simulink model "afe_rst_inv_psm_distributed_control_two_delays"  (R2026a)
settings: Solver=ode1be  StopTime=simlength  FixedStep=tc  MaxStep=Tc
values from neighbouring files (symbols this model uses):
  Amplitude_U = 1.16    [grid_fault_generator.m]
  Amplitude_V = Amplitude_U    (= 1.16)    [grid_fault_generator.m]
  Amplitude_W = Amplitude_U    (= 1.16)    [grid_fault_generator.m]
  end_time_LVRT = start_time_LVRT + error_length    [grid_fault_generator.m]
  Igrid_phase_normalization_factor = 270*sqrt(2)    [grid_emulator.m]
  omega_grid_emulator_nom = w_grid    (= 314.159265359)    [grid_emulator.m]
  omega_grid_nom = w_grid    (= 314.159265359)    [grid_emulator.m]
  t_ramp = 20e-3    (= 0.02)    [grid_fault_generator.m]
  ugrid_factor = 1    [grid_emulator.m]
  V_phase_normalization_factor = Vgrid_phase_normalization_factor    [grid_emulator.m]
  Vdc_bez = 1070    [grid_emulator.m]
  Vemu_ref_norm = Vemu_ref * sqrt(2) / V_phase_normalization_factor    [grid_emulator.m]
  vn_eta_pu = 0    [grid_emulator.m]
  vn_xi_pu = 0    [grid_emulator.m]
  vp_xi_pu = 1    [grid_emulator.m]
undefined symbols (not defined in the file or in its folder): Adrso, Aresd, Bresd, CFi, CFu, Cresd, Crso, CTRPIFF_CLIP_RELEASE, dead_time_INV, emf_fb_p, emf_fb_p_ccaller_1, emf_fb_p_ccaller_2, emf_p, emf_p_ccaller_1, emf_p_ccaller_2, fPWM_INV, g0_161Hz, g0_500Hz, g1_161Hz, g1_500Hz, i_grid_neg_eta_lim, i_grid_neg_eta_red_lim, i_grid_neg_xi_lim, i_grid_neg_xi_red_lim, i_grid_pos_eta_lim, i_grid_pos_eta_red_lim, ibez, id_lim, ieta_neg_ref_lim, ieta_pos_ref_lim, iq_lim, ixi_pos_ref_lim, Jm_norm, k_frt_ref, kg, ki_afe, ki_i, ki_id, ki_iq, ki_rc_neg_grid, ki_rc_pos_grid, ki_vs, ki_w, kp_afe, kp_i, kp_id, kp_iq, kp_rc_neg_grid, kp_rc_pos_grid, kp_vs, kp_w, kw, l1, l2, Lalpha_norm, Ld_norm, Ldrso, Lq_norm, Ls_norm, luenberger_l1 ... (+30)
libraries: fl_lib x146, nesl_utility x62, simulink x8, cstblocks_lti x7, sl_discontinuities x3, single_phase_transformer_lib x3, flexshaft_lib x1, permanent_magnet_synchronous_machine x1
(part 9 of 14)

== system afe_rst_inv_psm_distributed_control_two_delays/INV-Modular/inv_leg_w/driver_board_w/voltage-current-acquisition/usu_fieldbus ==
  us : Inport
  Unit Delay : UnitDelay  SampleTime=ts_inv
  Unit Delay1 : UnitDelay  SampleTime=ts_inv
  Zero-Order Hold : ZeroOrderHold  SampleTime=ts_inv
  us_fb : Outport
  wires:
  Zero-Order Hold/1 -> Unit Delay/1
  us/1 -> Zero-Order Hold/1
  Unit Delay/1 -> Unit Delay1/1
  Unit Delay1/1 -> us_fb/1

== system afe_rst_inv_psm_distributed_control_two_delays/INV-Modular/inv_leg_w/driver_board_w/voltage-current-acquisition/usv_ctrl_fieldbus ==
  u_ctrl : Inport
  Unit Delay : UnitDelay  SampleTime=ts_inv
  Unit Delay1 : UnitDelay  SampleTime=ts_inv
  Zero-Order Hold : ZeroOrderHold  SampleTime=ts_inv
  u_ctrl_fb : Outport
  wires:
  Zero-Order Hold/1 -> Unit Delay/1
  u_ctrl/1 -> Zero-Order Hold/1
  Unit Delay/1 -> Unit Delay1/1
  Unit Delay1/1 -> u_ctrl_fb/1

== system afe_rst_inv_psm_distributed_control_two_delays/INV-Modular/inv_leg_w/driver_board_w/voltage-current-acquisition/usv_fieldbus ==
  us : Inport
  Unit Delay : UnitDelay  SampleTime=ts_inv
  Unit Delay1 : UnitDelay  SampleTime=ts_inv
  Zero-Order Hold : ZeroOrderHold  SampleTime=ts_inv
  us_fb : Outport
  wires:
  Zero-Order Hold/1 -> Unit Delay/1
  us/1 -> Zero-Order Hold/1
  Unit Delay/1 -> Unit Delay1/1
  Unit Delay1/1 -> us_fb/1

== system afe_rst_inv_psm_distributed_control_two_delays/INV-Modular/inv_leg_w/driver_board_w/voltage-current-acquisition/usw_measure_and_normalization ==
  us : Inport
  Gain : Gain  Gain=1/ubez
  Quantizer : Quantizer  QuantizationInterval=CurrentQuantization
  Unit Delay : UnitDelay  SampleTime=ts_afe
  Zero-Order Hold : ZeroOrderHold  SampleTime=ts_afe
  us_pu : Outport
  wires:
  Quantizer/1 -> Zero-Order Hold/1
  Gain/1 -> us_pu/1
  Zero-Order Hold/1 -> Unit Delay/1
  Unit Delay/1 -> Gain/1
  us/1 -> Quantizer/1

== system afe_rst_inv_psm_distributed_control_two_delays/INV-Modular/inv_leg_w/modulator/sv_pwm/modulator ==
  w : Inport
  Bus Creator : BusCreator  Inputs=2
  PWM generator : Subsystem  mask{f=fPWM_INV, ph=0, m_up=0.98, m_low=0.02, dead_time=dead_time_INV, vg_firing=15, polarity=1}
      mask prompts: f "Frequency"; ph "Phase"; m_up "Max Input Modulation Value"; m_low "Min Input Modulation Value"; dead_time "Dead Time"; vg_firing "Gate Voltage"
  firing_gates : Outport
  wires:
  PWM generator/2(m2) -> Bus Creator/2  "pwm_w_bottom"
  PWM generator/1(m1) -> Bus Creator/1  "pwm_w_top"
  Bus Creator/1 -> firing_gates/1
  w/1 -> PWM generator/1(m_index)

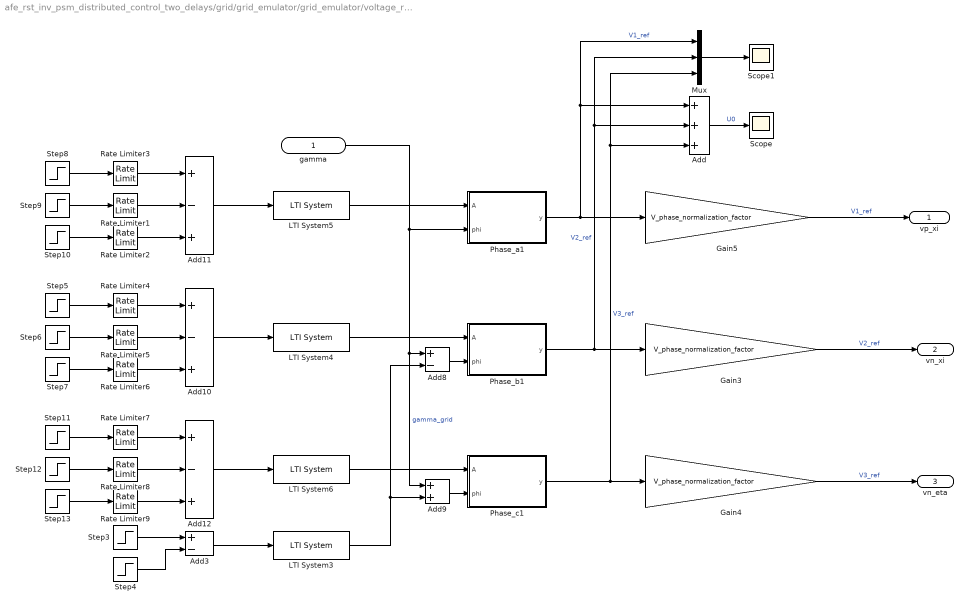
== system afe_rst_inv_psm_distributed_control_two_delays/grid/grid_emulator/grid_emulator/voltage_reference/Grid: Voltage-Source in abc ==
  gamma : Inport
  Add : Sum  Inputs=+++
  Add10 : Sum  Inputs=+-+
  Add11 : Sum  Inputs=+-+
  Add12 : Sum  Inputs=+-+
  Add3 : Sum  Inputs=+-
  Add8 : Sum  Inputs=+-
  Add9 : Sum
  Gain3 : Gain  Gain=V_phase_normalization_factor
  Gain4 : Gain  Gain=V_phase_normalization_factor
  Gain5 : Gain  Gain=V_phase_normalization_factor
  LTI System{3..6} (4 alike) : cstblocks_lti/LTI System  sys=LVRT_flt_ss_c  IC=[0]  PadeOrder=0
  Mux : Mux  Inputs=3
  Phase_a1 : MATLAB Function  TreatAsAtomicUnit=on
  Phase_b1 : MATLAB Function  TreatAsAtomicUnit=on
  Phase_c1 : MATLAB Function  TreatAsAtomicUnit=on
  Rate Limiter{1..9} (9 alike) : RateLimiter  RisingSlewLimit=Vemu_ref_norm/t_ramp  FallingSlewLimit=-Vemu_ref_norm/t_ramp  SampleTimeMode=inherited
  Scope : Scope
      settings: SampleTime=tc  ActiveDisplayYMinimum=-1.1E-15  ActiveDisplayYMaximum=9E-16
  Scope1 : Scope
      settings: SampleTime=tc  ActiveDisplayYMinimum=-1.24491  ActiveDisplayYMaximum=1.24491
  Step10 : Step  Time=end_time_LVRT  FinalValue=Vemu_ref_norm*(1-Amplitude_U)  SampleTime=0
  Step11 : Step  Time=0  FinalValue=Vemu_ref_norm  SampleTime=0
  Step12 : Step  Time=start_time_LVRT  FinalValue=Vemu_ref_norm*(1-Amplitude_W)  SampleTime=0
  Step13 : Step  Time=end_time_LVRT  FinalValue=Vemu_ref_norm*(1-Amplitude_W)  SampleTime=0
  Step3 : Step  Time=start_time_LVRT  FinalValue=Phase_shift  SampleTime=0
  Step4 : Step  Time=end_time_LVRT  FinalValue=Phase_shift  SampleTime=0
  Step5 : Step  Time=0  FinalValue=Vemu_ref_norm  SampleTime=0
  Step6 : Step  Time=start_time_LVRT  FinalValue=Vemu_ref_norm*(1-Amplitude_V)  SampleTime=0
  Step7 : Step  Time=end_time_LVRT  FinalValue=Vemu_ref_norm*(1-Amplitude_V)  SampleTime=0
  Step8 : Step  Time=0  FinalValue=Vemu_ref_norm  SampleTime=0
  Step9 : Step  Time=start_time_LVRT  FinalValue=Vemu_ref_norm*(1-Amplitude_U)  SampleTime=0
  vp_xi : Outport  VectorParamsAs1DForOutWhenUnconnected=off
  vn_xi : Outport  Port=2  VectorParamsAs1DForOutWhenUnconnected=off
  vn_eta : Outport  Port=3  VectorParamsAs1DForOutWhenUnconnected=off
  wires:
  Phase_c1/1(y) -> Mux/3, Add/3, Gain4/1  "V3_ref"
  LTI System6/1 -> Phase_c1/1(A)
  gamma/1 -> Add9/1, Add8/1, Phase_a1/2(phi)  "gamma_grid"
  Add9/1 -> Phase_c1/2(phi)
  Add8/1 -> Phase_b1/2(phi)
  Phase_b1/1(y) -> Mux/2, Add/2, Gain3/1  "V2_ref"
  Phase_a1/1(y) -> Mux/1, Add/1, Gain5/1  "V1_ref"
  LTI System4/1 -> Phase_b1/1(A)
  Step5/1 -> Rate Limiter4/1
  Step6/1 -> Rate Limiter5/1
  Step7/1 -> Rate Limiter6/1
  Add10/1 -> LTI System4/1
  Step8/1 -> Rate Limiter3/1
  Add11/1 -> LTI System5/1
  Step9/1 -> Rate Limiter1/1
  Step10/1 -> Rate Limiter2/1
  LTI System5/1 -> Phase_a1/1(A)
  Add12/1 -> LTI System6/1
  Rate Limiter3/1 -> Add11/1
  Rate Limiter1/1 -> Add11/2
  Rate Limiter2/1 -> Add11/3
  Rate Limiter4/1 -> Add10/1
  Rate Limiter5/1 -> Add10/2
  Rate Limiter6/1 -> Add10/3
  Step12/1 -> Rate Limiter8/1
  Rate Limiter8/1 -> Add12/2
  Step13/1 -> Rate Limiter9/1
  Rate Limiter9/1 -> Add12/3
  Step11/1 -> Rate Limiter7/1
  Rate Limiter7/1 -> Add12/1
  Gain5/1 -> vp_xi/1  "V1_ref"
  Gain3/1 -> vn_xi/1  "V2_ref"
  Gain4/1 -> vn_eta/1  "V3_ref"
  Add3/1 -> LTI System3/1
  Step3/1 -> Add3/1
  Step4/1 -> Add3/2
  LTI System3/1 -> Add9/2, Add8/2
  Add/1 -> Scope/1  "U0"
  Mux/1 -> Scope1/1

== system afe_rst_inv_psm_distributed_control_two_delays/mainboard_afe/dq_pll/pll_stageA/sequences/alphabeta2xieta ==
  alpha : Inport
  beta : Inport  Port=2
  gamma : Inport  Port=3
  alphabeta2xieta_neg : MATLAB Function  TreatAsAtomicUnit=on  SystemSampleTime=ts_afe
  alphabeta2xieta_pos : MATLAB Function  TreatAsAtomicUnit=on  SystemSampleTime=ts_afe
  xi : Outport
  eta : Outport  Port=2
  Out3 : Outport  Port=3
  Out4 : Outport  Port=4
  wires:
  alpha/1 -> alphabeta2xieta_neg/1(alpha), alphabeta2xieta_pos/1(alpha)  "u_grid_alpha"
  beta/1 -> alphabeta2xieta_neg/2(beta), alphabeta2xieta_pos/2(beta)  "u_grid_beta"
  gamma/1 -> alphabeta2xieta_neg/3(gamma), alphabeta2xieta_pos/3(gamma)  "gamma_grid"
  alphabeta2xieta_pos/1(xi) -> xi/1  "u_grid_pos_xi"
  alphabeta2xieta_pos/2(eta) -> eta/1  "u_grid_pos_eta"
  alphabeta2xieta_neg/1(xi) -> Out3/1  "u_grid_neg_xi"
  alphabeta2xieta_neg/2(eta) -> Out4/1  "u_grid_neg_eta"

== system afe_rst_inv_psm_distributed_control_two_delays/AFE-Modular/afe_leg_a/driver_board_a/current_ctrl/phase_current_control/phase-current-control-dba ==
  In1 : Inport
  is_abc : Inport  Port=2
  Add : Sum
  Add1 : Sum
  Cresd./Tcontrol new1 : Gain  Gain=Cresd  Multiplication=Matrix(K*u)
  Gain : Gain  Gain=kp_afe
  Gain1 : Gain  Gain=ki_afe
  Gain2 : Gain  Gain=Bresd  Multiplication=Matrix(K*u)
  Gain3 : Gain  Gain=Aresd  Multiplication=Matrix(K*u)
  Sum : Sum  Inputs=|+-
  Sum2 : Sum  Inputs=|++  SaturateOnIntegerOverflow=on
  Unit Delay : UnitDelay  InitialCondition=[0 0]  SampleTime=ts_afe
  Out1 : Outport
  wires:
  Cresd./Tcontrol new1/1 -> Add/2  "y(k)"
  Gain3/1 -> Sum2/2
  Sum2/1 -> Unit Delay/1  "x(k+1)"
  Unit Delay/1 -> Cresd./Tcontrol new1/1, Gain3/1  "x(k)"
  Gain2/1 -> Sum2/1
  Gain1/1 -> Gain2/1  "u(k)"
  Gain/1 -> Add/1
  Sum/1 -> Gain/1, Gain1/1
  is_abc/1 -> Sum/2  "isa"
  In1/1 -> Sum/1  "isa_ref"
  Add/1 -> Add1/1  "u_ctrl_a"
  [uga_pu_dba_flt] -> Add1/2
  Add1/1 -> Out1/1  "u_ctrl_a"

== system afe_rst_inv_psm_distributed_control_two_delays/AFE-Modular/afe_leg_a/driver_board_a/dq_pll/pll_stageA/sequences ==
  u_grid_alpha : Inport
  u_grid_beta : Inport  Port=2
  gamma_grid : Inport  Port=3
  alphabeta2xieta : Subsystem
  u_grid_pos_xi : Outport
  u_grid_pos_eta : Outport  Port=2
  wires:
  alphabeta2xieta/1(xi) -> u_grid_pos_xi/1  "u_grid_pos_xi"
  alphabeta2xieta/2(eta) -> u_grid_pos_eta/1  "u_grid_pos_eta"
  u_grid_alpha/1 -> alphabeta2xieta/1(alpha)  "u_grid_alpha"
  u_grid_beta/1 -> alphabeta2xieta/2(beta)  "u_grid_beta"
  gamma_grid/1 -> alphabeta2xieta/3(gamma)  "gamma_grid"

== system afe_rst_inv_psm_distributed_control_two_delays/AFE-Modular/afe_leg_a/driver_board_a/dq_pll/pll_stageA/transformation ==
  ug_a : Inport
  ug_b : Inport  Port=2
  ug_c : Inport  Port=3
  abc2alphabeta : MATLAB Function  TreatAsAtomicUnit=on  SystemSampleTime=ts_afe
  u_500Hz_flt : Subsystem
  ug_alpha : Outport  VectorParamsAs1DForOutWhenUnconnected=off
  ug_beta : Outport  Port=2  VectorParamsAs1DForOutWhenUnconnected=off
  tag scope: uga_pu_dba_flt=global
  wires:
  abc2alphabeta/2(beta) -> ug_beta/1  "u_grid_beta"
  abc2alphabeta/1(alpha) -> ug_alpha/1  "u_grid_alpha"
  ug_c/1 -> abc2alphabeta/3(c)
  ug_b/1 -> abc2alphabeta/2(b)
  u_500Hz_flt/1(output) -> [uga_pu_dba_flt]
  ug_a/1 -> u_500Hz_flt/1(input), abc2alphabeta/1(a)

== system afe_rst_inv_psm_distributed_control_two_delays/AFE-Modular/afe_leg_a/modulator/sv_pwm/modulator/PWM generator 1 ==
  m_index : Inport
  Constant : Constant  Value=dead_time*f
  Constant1 : Constant
  Data Type Conversion1 : DataTypeConversion
  Data Type Conversion2 : DataTypeConversion
  Gain : Gain  Gain=1/(pi/2)
  Gain1 : Gain  Gain=1/2
  Gain2 : Gain  Gain=vg_firing
  Gain3 : Gain  Gain=vg_firing
  Gain4 : Gain  Gain=polarity
  Gain5 : Gain  Gain=polarity
  Hit Crossing : HitCross  Commented=on  ShowOutputPort=off
  Hit Crossing1 : HitCross  Commented=on  ShowOutputPort=off
  Relational Operator1 : RelationalOperator  Operator=<=  InputSameDT=off
  Relational Operator2 : RelationalOperator  Operator=<=  InputSameDT=off
  Saturation1 : Saturate  UpperLimit=m_up  LowerLimit=m_low
  Sine Wave : Sin  Frequency=f*2*pi  Phase=-pi/2+ph  SampleTime=0
  Sum : Sum  Inputs=|++  SaturateOnIntegerOverflow=on
  Sum1 : Sum  Inputs=-+|  SaturateOnIntegerOverflow=on
  Sum2 : Sum  Inputs=|++
  Trigonometric Function1 : Trigonometry  Operator=asin
  m1 : Outport
  m2 : Outport  Port=2
  wires:
  Relational Operator1/1 -> Data Type Conversion1/1
  m_index/1 -> Saturation1/1
  Relational Operator2/1 -> Data Type Conversion2/1
  Data Type Conversion2/1 -> Gain3/1, Hit Crossing1/1
  Constant/1 -> Sum/2, Sum1/1
  Saturation1/1 -> Sum/1, Sum1/2
  Sum/1 -> Relational Operator1/1
  Sum1/1 -> Relational Operator2/2
  Sine Wave/1 -> Trigonometric Function1/1
  Constant1/1 -> Sum2/2
  Trigonometric Function1/1 -> Gain/1
  Gain/1 -> Sum2/1
  Sum2/1 -> Gain1/1
  Gain1/1 -> Relational Operator2/1, Relational Operator1/2
  Data Type Conversion1/1 -> Hit Crossing/1, Gain2/1
  Gain2/1 -> Gain4/1
  Gain3/1 -> Gain5/1
  Gain4/1 -> m1/1
  Gain5/1 -> m2/1

== system afe_rst_inv_psm_distributed_control_two_delays/AFE-Modular/afe_leg_a/modulator/sv_pwm/modulator/PWM generator 2 ==
  m_index : Inport
  Constant : Constant  Value=dead_time*f
  Constant1 : Constant
  Data Type Conversion1 : DataTypeConversion
  Data Type Conversion2 : DataTypeConversion
  Gain : Gain  Gain=1/(pi/2)
  Gain1 : Gain  Gain=1/2
  Gain2 : Gain  Gain=vg_firing
  Gain3 : Gain  Gain=vg_firing
  Gain4 : Gain  Gain=polarity
  Gain5 : Gain  Gain=polarity
  Hit Crossing : HitCross  Commented=on  ShowOutputPort=off
  Hit Crossing1 : HitCross  Commented=on  ShowOutputPort=off
  Relational Operator1 : RelationalOperator  Operator=<=  InputSameDT=off
  Relational Operator2 : RelationalOperator  Operator=<=  InputSameDT=off
  Saturation1 : Saturate  UpperLimit=m_up  LowerLimit=m_low
  Sine Wave : Sin  Frequency=f*2*pi  Phase=-pi/2+ph  SampleTime=0
  Sum : Sum  Inputs=|++  SaturateOnIntegerOverflow=on
  Sum1 : Sum  Inputs=-+|  SaturateOnIntegerOverflow=on
  Sum2 : Sum  Inputs=|++
  Trigonometric Function1 : Trigonometry  Operator=asin
  m1 : Outport
  m2 : Outport  Port=2
  wires:
  Gain5/1 -> m2/1
  Gain4/1 -> m1/1
  Gain3/1 -> Gain5/1
  Gain2/1 -> Gain4/1
  Data Type Conversion1/1 -> Gain2/1, Hit Crossing/1
  Gain1/1 -> Relational Operator1/2, Relational Operator2/1
  Sum2/1 -> Gain1/1
  Gain/1 -> Sum2/1
  Trigonometric Function1/1 -> Gain/1
  Constant1/1 -> Sum2/2
  Sine Wave/1 -> Trigonometric Function1/1
  Sum1/1 -> Relational Operator2/2
  Sum/1 -> Relational Operator1/1
  Saturation1/1 -> Sum1/2, Sum/1
  Constant/1 -> Sum1/1, Sum/2
  Data Type Conversion2/1 -> Hit Crossing1/1, Gain3/1
  Relational Operator2/1 -> Data Type Conversion2/1
  m_index/1 -> Saturation1/1
  Relational Operator1/1 -> Data Type Conversion1/1

== system afe_rst_inv_psm_distributed_control_two_delays/AFE-Modular/afe_leg_a/modulator/sv_pwm/modulator/PWM generator 3 ==
  m_index : Inport
  Constant : Constant  Value=dead_time*f
  Constant1 : Constant
  Data Type Conversion1 : DataTypeConversion
  Data Type Conversion2 : DataTypeConversion
  Gain : Gain  Gain=1/(pi/2)
  Gain1 : Gain  Gain=1/2
  Gain2 : Gain  Gain=vg_firing
  Gain3 : Gain  Gain=vg_firing
  Gain4 : Gain  Gain=polarity
  Gain5 : Gain  Gain=polarity
  Hit Crossing : HitCross  Commented=on  ShowOutputPort=off
  Hit Crossing1 : HitCross  Commented=on  ShowOutputPort=off
  Relational Operator1 : RelationalOperator  Operator=<=  InputSameDT=off
  Relational Operator2 : RelationalOperator  Operator=<=  InputSameDT=off
  Saturation1 : Saturate  UpperLimit=m_up  LowerLimit=m_low
  Sine Wave : Sin  Frequency=f*2*pi  Phase=-pi/2+ph  SampleTime=0
  Sum : Sum  Inputs=|++  SaturateOnIntegerOverflow=on
  Sum1 : Sum  Inputs=-+|  SaturateOnIntegerOverflow=on
  Sum2 : Sum  Inputs=|++
  Trigonometric Function1 : Trigonometry  Operator=asin
  m1 : Outport
  m2 : Outport  Port=2
  wires:
  Relational Operator1/1 -> Data Type Conversion1/1
  m_index/1 -> Saturation1/1
  Relational Operator2/1 -> Data Type Conversion2/1
  Data Type Conversion2/1 -> Gain3/1, Hit Crossing1/1
  Constant/1 -> Sum/2, Sum1/1
  Saturation1/1 -> Sum/1, Sum1/2
  Sum/1 -> Relational Operator1/1
  Sum1/1 -> Relational Operator2/2
  Sine Wave/1 -> Trigonometric Function1/1
  Constant1/1 -> Sum2/2
  Trigonometric Function1/1 -> Gain/1
  Gain/1 -> Sum2/1
  Sum2/1 -> Gain1/1
  Gain1/1 -> Relational Operator2/1, Relational Operator1/2
  Data Type Conversion1/1 -> Hit Crossing/1, Gain2/1
  Gain2/1 -> Gain4/1
  Gain3/1 -> Gain5/1
  Gain4/1 -> m1/1
  Gain5/1 -> m2/1

== system afe_rst_inv_psm_distributed_control_two_delays/AFE-Modular/afe_leg_b/driver_board_b/current_ctrl/phase_current_control/phase-current-control-dbb ==
  In1 : Inport
  is_abc : Inport  Port=2
  Add : Sum
  Add1 : Sum
  Cresd./Tcontrol new1 : Gain  Gain=Cresd  Multiplication=Matrix(K*u)
  Gain : Gain  Gain=kp_afe
  Gain1 : Gain  Gain=ki_afe
  Gain2 : Gain  Gain=Bresd  Multiplication=Matrix(K*u)
  Gain3 : Gain  Gain=Aresd  Multiplication=Matrix(K*u)
  Sum : Sum  Inputs=|+-
  Sum2 : Sum  Inputs=|++  SaturateOnIntegerOverflow=on
  Unit Delay : UnitDelay  InitialCondition=[0 0]  SampleTime=ts_afe
  Out1 : Outport
  wires:
  Cresd./Tcontrol new1/1 -> Add/2  "y(k)"
  Gain3/1 -> Sum2/2
  Sum2/1 -> Unit Delay/1  "x(k+1)"
  Unit Delay/1 -> Cresd./Tcontrol new1/1, Gain3/1  "x(k)"
  Gain2/1 -> Sum2/1
  Gain1/1 -> Gain2/1  "u(k)"
  Gain/1 -> Add/1
  Sum/1 -> Gain/1, Gain1/1
  is_abc/1 -> Sum/2  "isb"
  In1/1 -> Sum/1  "isb_ref"
  [ugb_pu_dbb_flt] -> Add1/2
  Add/1 -> Add1/1  "u_ctrl_b"
  Add1/1 -> Out1/1  "u_ctrl_b"

== system afe_rst_inv_psm_distributed_control_two_delays/AFE-Modular/afe_leg_b/driver_board_b/dq_pll/pll_stageA/mormalization_and_transformation ==
  ug_a : Inport
  ug_b : Inport  Port=2
  ug_c : Inport  Port=3
  abc2alphabeta : MATLAB Function  TreatAsAtomicUnit=on  SystemSampleTime=ts_afe
  u_500Hz_flt : Subsystem
  ug_alpha : Outport  VectorParamsAs1DForOutWhenUnconnected=off
  ug_beta : Outport  Port=2  VectorParamsAs1DForOutWhenUnconnected=off
  tag scope: ugb_pu_dbb_flt=global
  wires:
  abc2alphabeta/2(beta) -> ug_beta/1  "u_grid_beta"
  abc2alphabeta/1(alpha) -> ug_alpha/1  "u_grid_alpha"
  ug_c/1 -> abc2alphabeta/3(c)
  ug_b/1 -> u_500Hz_flt/1(input), abc2alphabeta/2(b)
  u_500Hz_flt/1(output) -> [ugb_pu_dbb_flt]
  ug_a/1 -> abc2alphabeta/1(a)

== system afe_rst_inv_psm_distributed_control_two_delays/AFE-Modular/afe_leg_b/driver_board_b/dq_pll/pll_stageA/sequences ==
  u_grid_alpha : Inport
  u_grid_beta : Inport  Port=2
  gamma_grid : Inport  Port=3
  alphabeta2xieta : Subsystem
  u_grid_pos_xi : Outport
  u_grid_pos_eta : Outport  Port=2
  wires:
  alphabeta2xieta/1(xi) -> u_grid_pos_xi/1  "u_grid_pos_xi"
  alphabeta2xieta/2(eta) -> u_grid_pos_eta/1  "u_grid_pos_eta"
  u_grid_alpha/1 -> alphabeta2xieta/1(alpha)  "u_grid_alpha"
  u_grid_beta/1 -> alphabeta2xieta/2(beta)  "u_grid_beta"
  gamma_grid/1 -> alphabeta2xieta/3(gamma)  "gamma_grid"

== system afe_rst_inv_psm_distributed_control_two_delays/AFE-Modular/afe_leg_b/modulator/sv_pwm/modulator/PWM generator 1 ==
  m_index : Inport
  Constant : Constant  Value=dead_time*f
  Constant1 : Constant
  Data Type Conversion1 : DataTypeConversion
  Data Type Conversion2 : DataTypeConversion
  Gain : Gain  Gain=1/(pi/2)
  Gain1 : Gain  Gain=1/2
  Gain2 : Gain  Gain=vg_firing
  Gain3 : Gain  Gain=vg_firing
  Gain4 : Gain  Gain=polarity
  Gain5 : Gain  Gain=polarity
  Hit Crossing : HitCross  Commented=on  ShowOutputPort=off
  Hit Crossing1 : HitCross  Commented=on  ShowOutputPort=off
  Relational Operator1 : RelationalOperator  Operator=<=  InputSameDT=off
  Relational Operator2 : RelationalOperator  Operator=<=  InputSameDT=off
  Saturation1 : Saturate  UpperLimit=m_up  LowerLimit=m_low
  Sine Wave : Sin  Frequency=f*2*pi  Phase=-pi/2+ph  SampleTime=0
  Sum : Sum  Inputs=|++  SaturateOnIntegerOverflow=on
  Sum1 : Sum  Inputs=-+|  SaturateOnIntegerOverflow=on
  Sum2 : Sum  Inputs=|++
  Trigonometric Function1 : Trigonometry  Operator=asin
  m1 : Outport
  m2 : Outport  Port=2
  wires:
  Gain5/1 -> m2/1
  Gain4/1 -> m1/1
  Gain3/1 -> Gain5/1
  Gain2/1 -> Gain4/1
  Data Type Conversion1/1 -> Gain2/1, Hit Crossing/1
  Gain1/1 -> Relational Operator1/2, Relational Operator2/1
  Sum2/1 -> Gain1/1
  Gain/1 -> Sum2/1
  Trigonometric Function1/1 -> Gain/1
  Constant1/1 -> Sum2/2
  Sine Wave/1 -> Trigonometric Function1/1
  Sum1/1 -> Relational Operator2/2
  Sum/1 -> Relational Operator1/1
  Saturation1/1 -> Sum1/2, Sum/1
  Constant/1 -> Sum1/1, Sum/2
  Data Type Conversion2/1 -> Hit Crossing1/1, Gain3/1
  Relational Operator2/1 -> Data Type Conversion2/1
  m_index/1 -> Saturation1/1
  Relational Operator1/1 -> Data Type Conversion1/1

== system afe_rst_inv_psm_distributed_control_two_delays/AFE-Modular/afe_leg_b/modulator/sv_pwm/modulator/PWM generator 2 ==
  m_index : Inport
  Constant : Constant  Value=dead_time*f
  Constant1 : Constant
  Data Type Conversion1 : DataTypeConversion
  Data Type Conversion2 : DataTypeConversion
  Gain : Gain  Gain=1/(pi/2)
  Gain1 : Gain  Gain=1/2
  Gain2 : Gain  Gain=vg_firing
  Gain3 : Gain  Gain=vg_firing
  Gain4 : Gain  Gain=polarity
  Gain5 : Gain  Gain=polarity
  Hit Crossing : HitCross  Commented=on  ShowOutputPort=off
  Hit Crossing1 : HitCross  Commented=on  ShowOutputPort=off
  Relational Operator1 : RelationalOperator  Operator=<=  InputSameDT=off
  Relational Operator2 : RelationalOperator  Operator=<=  InputSameDT=off
  Saturation1 : Saturate  UpperLimit=m_up  LowerLimit=m_low
  Sine Wave : Sin  Frequency=f*2*pi  Phase=-pi/2+ph  SampleTime=0
  Sum : Sum  Inputs=|++  SaturateOnIntegerOverflow=on
  Sum1 : Sum  Inputs=-+|  SaturateOnIntegerOverflow=on
  Sum2 : Sum  Inputs=|++
  Trigonometric Function1 : Trigonometry  Operator=asin
  m1 : Outport
  m2 : Outport  Port=2
  wires:
  Relational Operator1/1 -> Data Type Conversion1/1
  m_index/1 -> Saturation1/1
  Relational Operator2/1 -> Data Type Conversion2/1
  Data Type Conversion2/1 -> Gain3/1, Hit Crossing1/1
  Constant/1 -> Sum/2, Sum1/1
  Saturation1/1 -> Sum/1, Sum1/2
  Sum/1 -> Relational Operator1/1
  Sum1/1 -> Relational Operator2/2
  Sine Wave/1 -> Trigonometric Function1/1
  Constant1/1 -> Sum2/2
  Trigonometric Function1/1 -> Gain/1
  Gain/1 -> Sum2/1
  Sum2/1 -> Gain1/1
  Gain1/1 -> Relational Operator2/1, Relational Operator1/2
  Data Type Conversion1/1 -> Hit Crossing/1, Gain2/1
  Gain2/1 -> Gain4/1
  Gain3/1 -> Gain5/1
  Gain4/1 -> m1/1
  Gain5/1 -> m2/1

== system afe_rst_inv_psm_distributed_control_two_delays/AFE-Modular/afe_leg_b/modulator/sv_pwm/modulator/PWM generator 3 ==
  m_index : Inport
  Constant : Constant  Value=dead_time*f
  Constant1 : Constant
  Data Type Conversion1 : DataTypeConversion
  Data Type Conversion2 : DataTypeConversion
  Gain : Gain  Gain=1/(pi/2)
  Gain1 : Gain  Gain=1/2
  Gain2 : Gain  Gain=vg_firing
  Gain3 : Gain  Gain=vg_firing
  Gain4 : Gain  Gain=polarity
  Gain5 : Gain  Gain=polarity
  Hit Crossing : HitCross  Commented=on  ShowOutputPort=off
  Hit Crossing1 : HitCross  Commented=on  ShowOutputPort=off
  Relational Operator1 : RelationalOperator  Operator=<=  InputSameDT=off
  Relational Operator2 : RelationalOperator  Operator=<=  InputSameDT=off
  Saturation1 : Saturate  UpperLimit=m_up  LowerLimit=m_low
  Sine Wave : Sin  Frequency=f*2*pi  Phase=-pi/2+ph  SampleTime=0
  Sum : Sum  Inputs=|++  SaturateOnIntegerOverflow=on
  Sum1 : Sum  Inputs=-+|  SaturateOnIntegerOverflow=on
  Sum2 : Sum  Inputs=|++
  Trigonometric Function1 : Trigonometry  Operator=asin
  m1 : Outport
  m2 : Outport  Port=2
  wires:
  Gain5/1 -> m2/1
  Gain4/1 -> m1/1
  Gain3/1 -> Gain5/1
  Gain2/1 -> Gain4/1
  Data Type Conversion1/1 -> Gain2/1, Hit Crossing/1
  Gain1/1 -> Relational Operator1/2, Relational Operator2/1
  Sum2/1 -> Gain1/1
  Gain/1 -> Sum2/1
  Trigonometric Function1/1 -> Gain/1
  Constant1/1 -> Sum2/2
  Sine Wave/1 -> Trigonometric Function1/1
  Sum1/1 -> Relational Operator2/2
  Sum/1 -> Relational Operator1/1
  Saturation1/1 -> Sum1/2, Sum/1
  Constant/1 -> Sum1/1, Sum/2
  Data Type Conversion2/1 -> Hit Crossing1/1, Gain3/1
  Relational Operator2/1 -> Data Type Conversion2/1
  m_index/1 -> Saturation1/1
  Relational Operator1/1 -> Data Type Conversion1/1

== system afe_rst_inv_psm_distributed_control_two_delays/AFE-Modular/afe_leg_c/driver_board_c/current_ctrl/phase_current_control/phase-current-control-dbc ==
  In1 : Inport
  is_abc : Inport  Port=2
  Add : Sum
  Add1 : Sum
  Cresd./Tcontrol new1 : Gain  Gain=Cresd  Multiplication=Matrix(K*u)
  Gain : Gain  Gain=kp_afe
  Gain1 : Gain  Gain=ki_afe
  Gain2 : Gain  Gain=Bresd  Multiplication=Matrix(K*u)
  Gain3 : Gain  Gain=Aresd  Multiplication=Matrix(K*u)
  Sum : Sum  Inputs=|+-
  Sum2 : Sum  Inputs=|++  SaturateOnIntegerOverflow=on
  Unit Delay : UnitDelay  InitialCondition=[0 0]  SampleTime=ts_afe
  Out1 : Outport
  wires:
  Cresd./Tcontrol new1/1 -> Add/2  "y(k)"
  Gain3/1 -> Sum2/2
  Sum2/1 -> Unit Delay/1  "x(k+1)"
  Unit Delay/1 -> Cresd./Tcontrol new1/1, Gain3/1  "x(k)"
  Gain2/1 -> Sum2/1
  Gain1/1 -> Gain2/1  "u(k)"
  Gain/1 -> Add/1
  Sum/1 -> Gain/1, Gain1/1
  is_abc/1 -> Sum/2  "isb"
  In1/1 -> Sum/1  "isb_ref"
  [ugc_pu_dbc_flt] -> Add1/2
  Add/1 -> Add1/1  "u_ctrl_c"
  Add1/1 -> Out1/1  "u_ctrl_c"

== system afe_rst_inv_psm_distributed_control_two_delays/AFE-Modular/afe_leg_c/driver_board_c/dq_pll/pll_stageA/mormalization_and_transformation ==
  ug_a : Inport
  ug_b : Inport  Port=2
  ug_c : Inport  Port=3
  abc2alphabeta : MATLAB Function  TreatAsAtomicUnit=on  SystemSampleTime=ts_afe
  u_500Hz_flt : Subsystem
  ug_alpha : Outport  VectorParamsAs1DForOutWhenUnconnected=off
  ug_beta : Outport  Port=2  VectorParamsAs1DForOutWhenUnconnected=off
  tag scope: ugc_pu_dbc_flt=global
  wires:
  abc2alphabeta/2(beta) -> ug_beta/1  "u_grid_beta"
  abc2alphabeta/1(alpha) -> ug_alpha/1  "u_grid_alpha"
  u_500Hz_flt/1(output) -> [ugc_pu_dbc_flt]
  ug_c/1 -> u_500Hz_flt/1(input), abc2alphabeta/3(c)
  ug_b/1 -> abc2alphabeta/2(b)
  ug_a/1 -> abc2alphabeta/1(a)

== system afe_rst_inv_psm_distributed_control_two_delays/AFE-Modular/afe_leg_c/driver_board_c/dq_pll/pll_stageA/sequences ==
  u_grid_alpha : Inport
  u_grid_beta : Inport  Port=2
  gamma_grid : Inport  Port=3
  alphabeta2xieta : Subsystem
  u_grid_pos_xi : Outport
  u_grid_pos_eta : Outport  Port=2
  wires:
  alphabeta2xieta/1(xi) -> u_grid_pos_xi/1  "u_grid_pos_xi"
  alphabeta2xieta/2(eta) -> u_grid_pos_eta/1  "u_grid_pos_eta"
  u_grid_alpha/1 -> alphabeta2xieta/1(alpha)  "u_grid_alpha"
  u_grid_beta/1 -> alphabeta2xieta/2(beta)  "u_grid_beta"
  gamma_grid/1 -> alphabeta2xieta/3(gamma)  "gamma_grid"

== system afe_rst_inv_psm_distributed_control_two_delays/AFE-Modular/afe_leg_c/modulator/sv_pwm/modulator/PWM generator 1 ==
  m_index : Inport
  Constant : Constant  Value=dead_time*f
  Constant1 : Constant
  Data Type Conversion1 : DataTypeConversion
  Data Type Conversion2 : DataTypeConversion
  Gain : Gain  Gain=1/(pi/2)
  Gain1 : Gain  Gain=1/2
  Gain2 : Gain  Gain=vg_firing
  Gain3 : Gain  Gain=vg_firing
  Gain4 : Gain  Gain=polarity
  Gain5 : Gain  Gain=polarity
  Hit Crossing : HitCross  Commented=on  ShowOutputPort=off
  Hit Crossing1 : HitCross  Commented=on  ShowOutputPort=off
  Relational Operator1 : RelationalOperator  Operator=<=  InputSameDT=off
  Relational Operator2 : RelationalOperator  Operator=<=  InputSameDT=off
  Saturation1 : Saturate  UpperLimit=m_up  LowerLimit=m_low
  Sine Wave : Sin  Frequency=f*2*pi  Phase=-pi/2+ph  SampleTime=0
  Sum : Sum  Inputs=|++  SaturateOnIntegerOverflow=on
  Sum1 : Sum  Inputs=-+|  SaturateOnIntegerOverflow=on
  Sum2 : Sum  Inputs=|++
  Trigonometric Function1 : Trigonometry  Operator=asin
  m1 : Outport
  m2 : Outport  Port=2
  wires:
  Relational Operator1/1 -> Data Type Conversion1/1
  m_index/1 -> Saturation1/1
  Relational Operator2/1 -> Data Type Conversion2/1
  Data Type Conversion2/1 -> Gain3/1, Hit Crossing1/1
  Constant/1 -> Sum/2, Sum1/1
  Saturation1/1 -> Sum/1, Sum1/2
  Sum/1 -> Relational Operator1/1
  Sum1/1 -> Relational Operator2/2
  Sine Wave/1 -> Trigonometric Function1/1
  Constant1/1 -> Sum2/2
  Trigonometric Function1/1 -> Gain/1
  Gain/1 -> Sum2/1
  Sum2/1 -> Gain1/1
  Gain1/1 -> Relational Operator2/1, Relational Operator1/2
  Data Type Conversion1/1 -> Hit Crossing/1, Gain2/1
  Gain2/1 -> Gain4/1
  Gain3/1 -> Gain5/1
  Gain4/1 -> m1/1
  Gain5/1 -> m2/1

== system afe_rst_inv_psm_distributed_control_two_delays/AFE-Modular/afe_leg_c/modulator/sv_pwm/modulator/PWM generator 2 ==
  m_index : Inport
  Constant : Constant  Value=dead_time*f
  Constant1 : Constant
  Data Type Conversion1 : DataTypeConversion
  Data Type Conversion2 : DataTypeConversion
  Gain : Gain  Gain=1/(pi/2)
  Gain1 : Gain  Gain=1/2
  Gain2 : Gain  Gain=vg_firing
  Gain3 : Gain  Gain=vg_firing
  Gain4 : Gain  Gain=polarity
  Gain5 : Gain  Gain=polarity
  Hit Crossing : HitCross  Commented=on  ShowOutputPort=off
  Hit Crossing1 : HitCross  Commented=on  ShowOutputPort=off
  Relational Operator1 : RelationalOperator  Operator=<=  InputSameDT=off
  Relational Operator2 : RelationalOperator  Operator=<=  InputSameDT=off
  Saturation1 : Saturate  UpperLimit=m_up  LowerLimit=m_low
  Sine Wave : Sin  Frequency=f*2*pi  Phase=-pi/2+ph  SampleTime=0
  Sum : Sum  Inputs=|++  SaturateOnIntegerOverflow=on
  Sum1 : Sum  Inputs=-+|  SaturateOnIntegerOverflow=on
  Sum2 : Sum  Inputs=|++
  Trigonometric Function1 : Trigonometry  Operator=asin
  m1 : Outport
  m2 : Outport  Port=2
  wires:
  Gain5/1 -> m2/1
  Gain4/1 -> m1/1
  Gain3/1 -> Gain5/1
  Gain2/1 -> Gain4/1
  Data Type Conversion1/1 -> Gain2/1, Hit Crossing/1
  Gain1/1 -> Relational Operator1/2, Relational Operator2/1
  Sum2/1 -> Gain1/1
  Gain/1 -> Sum2/1
  Trigonometric Function1/1 -> Gain/1
  Constant1/1 -> Sum2/2
  Sine Wave/1 -> Trigonometric Function1/1
  Sum1/1 -> Relational Operator2/2
  Sum/1 -> Relational Operator1/1
  Saturation1/1 -> Sum1/2, Sum/1
  Constant/1 -> Sum1/1, Sum/2
  Data Type Conversion2/1 -> Hit Crossing1/1, Gain3/1
  Relational Operator2/1 -> Data Type Conversion2/1
  m_index/1 -> Saturation1/1
  Relational Operator1/1 -> Data Type Conversion1/1

== system afe_rst_inv_psm_distributed_control_two_delays/AFE-Modular/afe_leg_c/modulator/sv_pwm/modulator/PWM generator 3 ==
  m_index : Inport
  Constant : Constant  Value=dead_time*f
  Constant1 : Constant
  Data Type Conversion1 : DataTypeConversion
  Data Type Conversion2 : DataTypeConversion
  Gain : Gain  Gain=1/(pi/2)
  Gain1 : Gain  Gain=1/2
  Gain2 : Gain  Gain=vg_firing
  Gain3 : Gain  Gain=vg_firing
  Gain4 : Gain  Gain=polarity
  Gain5 : Gain  Gain=polarity
  Hit Crossing : HitCross  Commented=on  ShowOutputPort=off
  Hit Crossing1 : HitCross  Commented=on  ShowOutputPort=off
  Relational Operator1 : RelationalOperator  Operator=<=  InputSameDT=off
  Relational Operator2 : RelationalOperator  Operator=<=  InputSameDT=off
  Saturation1 : Saturate  UpperLimit=m_up  LowerLimit=m_low
  Sine Wave : Sin  Frequency=f*2*pi  Phase=-pi/2+ph  SampleTime=0
  Sum : Sum  Inputs=|++  SaturateOnIntegerOverflow=on
  Sum1 : Sum  Inputs=-+|  SaturateOnIntegerOverflow=on
  Sum2 : Sum  Inputs=|++
  Trigonometric Function1 : Trigonometry  Operator=asin
  m1 : Outport
  m2 : Outport  Port=2
  wires:
  Relational Operator1/1 -> Data Type Conversion1/1
  m_index/1 -> Saturation1/1
  Relational Operator2/1 -> Data Type Conversion2/1
  Data Type Conversion2/1 -> Gain3/1, Hit Crossing1/1
  Constant/1 -> Sum/2, Sum1/1
  Saturation1/1 -> Sum/1, Sum1/2
  Sum/1 -> Relational Operator1/1
  Sum1/1 -> Relational Operator2/2
  Sine Wave/1 -> Trigonometric Function1/1
  Constant1/1 -> Sum2/2
  Trigonometric Function1/1 -> Gain/1
  Gain/1 -> Sum2/1
  Sum2/1 -> Gain1/1
  Gain1/1 -> Relational Operator2/1, Relational Operator1/2
  Data Type Conversion1/1 -> Hit Crossing/1, Gain2/1
  Gain2/1 -> Gain4/1
  Gain3/1 -> Gain5/1
  Gain4/1 -> m1/1
  Gain5/1 -> m2/1

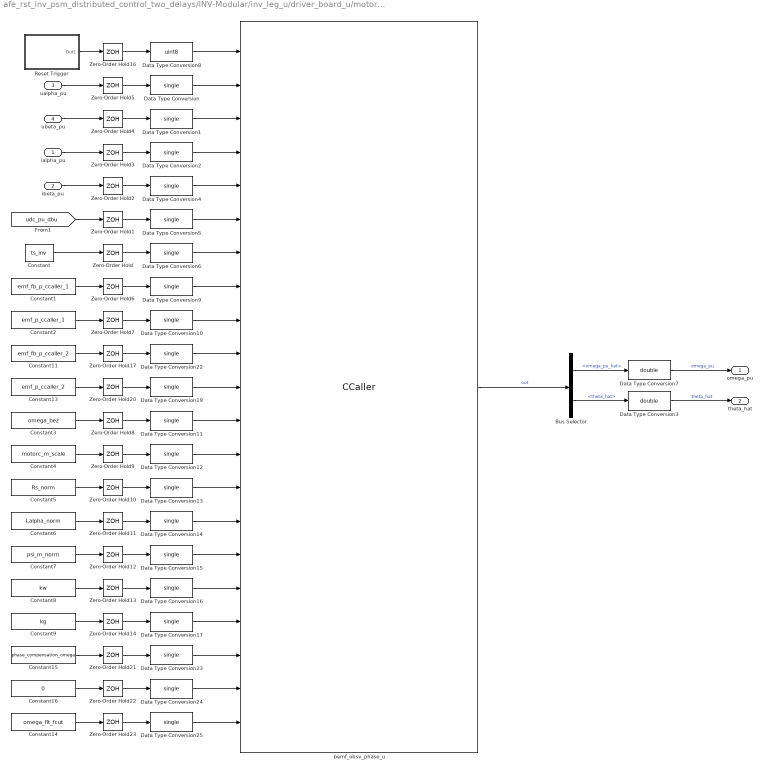
== system afe_rst_inv_psm_distributed_control_two_delays/INV-Modular/inv_leg_u/driver_board_u/motor_vector_control/bemf_observer/bemf_observer_ccaller ==
  ialpha_pu : Inport
  ibeta_pu : Inport  Port=2
  ualpha_pu : Inport  Port=3
  ubeta_pu : Inport  Port=4
  Bus Selector : BusSelector  OutputSignals=omega_pu_hat,theta_hat
  Constant : Constant  Value=ts_inv
  Constant1 : Constant  Value=emf_fb_p_ccaller_1
  Constant11 : Constant  Value=emf_fb_p_ccaller_2
  Constant13 : Constant  Value=emf_p_ccaller_2
  Constant14 : Constant  Value=omega_flt_fcut
  Constant15 : Constant  Value=phase_compensation_omega
  Constant16 : Constant  Value=0
  Constant2 : Constant  Value=emf_p_ccaller_1
  Constant3 : Constant  Value=omega_bez
  Constant4 : Constant  Value=motorc_m_scale
  Constant5 : Constant  Value=Rs_norm
  Constant6 : Constant  Value=Lalpha_norm
  Constant7 : Constant  Value=psi_m_norm
  Constant8 : Constant  Value=kw
  Constant9 : Constant  Value=kg
  Data Type Conversion{,1..2,4..6,9..17,19,22..25} (20 alike) : DataTypeConversion  OutDataTypeStr=single  SaturateOnIntegerOverflow=off  RndMeth=Floor
  Data Type Conversion3 : DataTypeConversion  OutDataTypeStr=double  SaturateOnIntegerOverflow=off  RndMeth=Floor
  Data Type Conversion7 : DataTypeConversion  OutDataTypeStr=double  SaturateOnIntegerOverflow=off  RndMeth=Floor
  Data Type Conversion8 : DataTypeConversion  OutDataTypeStr=uint8  SaturateOnIntegerOverflow=off  RndMeth=Floor
  Reset Trigger : Subsystem
  Zero-Order Hold{,1..14,16..17,20..23} (21 alike) : ZeroOrderHold  SampleTime=ts_inv
  bemf_obsv_phase_u : CCaller  FunctionName=bemf_obsv_process_simulink  PortSpecificationStruct="%)30     .    N\"8   8    (     @         %    \"    !8    !     0         %  0 \"0    $    _    07)G3F%M90  4&]R=$YA;64 4V-O<&4     26YD97@     5'EP90      4VEZ90      27-';&]B86P   X    P    !@    @    $          4    (     0    ,    !         !   P!O=70 #@   #     &    \"     0         !0    @    !     P    $         $  # &]U=  .    .     8    (    !          %    \"     $    &     0         0  ...(+12985 chars)"  SampleTime=ts_inv
  omega_pu : Outport
  theta_hat : Outport  Port=2
  wires:
  Zero-Order Hold21/1 -> Data Type Conversion23/1
  Zero-Order Hold22/1 -> Data Type Conversion24/1
  Constant15/1 -> Zero-Order Hold21/1
  Constant16/1 -> Zero-Order Hold22/1
  Constant14/1 -> Zero-Order Hold23/1
  Zero-Order Hold23/1 -> Data Type Conversion25/1
  Constant11/1 -> Zero-Order Hold17/1
  Zero-Order Hold17/1 -> Data Type Conversion22/1
  Zero-Order Hold20/1 -> Data Type Conversion19/1
  Constant13/1 -> Zero-Order Hold20/1
  Zero-Order Hold16/1 -> Data Type Conversion8/1
  Constant9/1 -> Zero-Order Hold14/1
  Constant8/1 -> Zero-Order Hold13/1
  Constant7/1 -> Zero-Order Hold12/1
  Constant6/1 -> Zero-Order Hold11/1
  Constant5/1 -> Zero-Order Hold10/1
  Constant4/1 -> Zero-Order Hold9/1
  Constant3/1 -> Zero-Order Hold8/1
  Constant2/1 -> Zero-Order Hold7/1
  Zero-Order Hold14/1 -> Data Type Conversion17/1
  Zero-Order Hold13/1 -> Data Type Conversion16/1
  Zero-Order Hold12/1 -> Data Type Conversion15/1
  Zero-Order Hold11/1 -> Data Type Conversion14/1
  Zero-Order Hold10/1 -> Data Type Conversion13/1
  Zero-Order Hold9/1 -> Data Type Conversion12/1
  Zero-Order Hold8/1 -> Data Type Conversion11/1
  Zero-Order Hold7/1 -> Data Type Conversion10/1
  Zero-Order Hold6/1 -> Data Type Conversion9/1
  Constant1/1 -> Zero-Order Hold6/1
  Data Type Conversion8/1 -> bemf_obsv_phase_u/1
  Reset Trigger/1(Out1) -> Zero-Order Hold16/1
  Data Type Conversion3/1 -> theta_hat/1  "theta_hat"
  Data Type Conversion7/1 -> omega_pu/1  "omega_pu"
  Bus Selector/1 -> Data Type Conversion7/1  "<omega_pu_hat>"
  Bus Selector/2 -> Data Type Conversion3/1  "<theta_hat>"
  ibeta_pu/1 -> Zero-Order Hold2/1
  ubeta_pu/1 -> Zero-Order Hold4/1
  ialpha_pu/1 -> Zero-Order Hold3/1
  ualpha_pu/1 -> Zero-Order Hold5/1
  Constant/1 -> Zero-Order Hold/1
  [udc_pu_dbu] -> Zero-Order Hold1/1
  Zero-Order Hold1/1 -> Data Type Conversion5/1
  Zero-Order Hold2/1 -> Data Type Conversion4/1
  Zero-Order Hold3/1 -> Data Type Conversion2/1
  Zero-Order Hold4/1 -> Data Type Conversion1/1
  Zero-Order Hold5/1 -> Data Type Conversion/1
  Zero-Order Hold/1 -> Data Type Conversion6/1
  Data Type Conversion2/1 -> bemf_obsv_phase_u/4
  Data Type Conversion4/1 -> bemf_obsv_phase_u/5
  Data Type Conversion1/1 -> bemf_obsv_phase_u/3
  bemf_obsv_phase_u/1 -> Bus Selector/1  "out"
  Data Type Conversion/1 -> bemf_obsv_phase_u/2
  Data Type Conversion5/1 -> bemf_obsv_phase_u/6
  Data Type Conversion23/1 -> bemf_obsv_phase_u/19
  Data Type Conversion24/1 -> bemf_obsv_phase_u/20
  Data Type Conversion25/1 -> bemf_obsv_phase_u/21
  Data Type Conversion17/1 -> bemf_obsv_phase_u/18
  Data Type Conversion16/1 -> bemf_obsv_phase_u/17
  Data Type Conversion15/1 -> bemf_obsv_phase_u/16
  Data Type Conversion14/1 -> bemf_obsv_phase_u/15
  Data Type Conversion13/1 -> bemf_obsv_phase_u/14
  Data Type Conversion12/1 -> bemf_obsv_phase_u/13
  Data Type Conversion11/1 -> bemf_obsv_phase_u/12
  Data Type Conversion19/1 -> bemf_obsv_phase_u/11
  Data Type Conversion22/1 -> bemf_obsv_phase_u/10
  Data Type Conversion10/1 -> bemf_obsv_phase_u/9
  Data Type Conversion9/1 -> bemf_obsv_phase_u/8
  Data Type Conversion6/1 -> bemf_obsv_phase_u/7
